simulink model "Testbed_R1"  (R2025a)
settings: Solver=ode1  StartTime=0.0  StopTime=TSTOP_R1  FixedStep=2e-6  RelTol=1e-3
undefined symbols (not defined in the file or in its folder): G_R1, Ion, Lithium, MODE_R1
libraries: spsSeriesRLCBranchLib x8, simulink x4, spsGroundLib x4, spsMosfetLib x4, spsControlledVoltageSourceLib x3, spsCurrentMeasurementLib x3, spsVoltageMeasurementLib x3, spsBatteryLib x1, spsThreePhaseSeriesRLCBranchLib x1, spsThreePhaseVIMeasurementLib x1, spsPVArrayLib x1, spsPWMGenerator2LevelLib x1
settings Model: Creator=ASUS  LastModifiedBy=ASUS
settings DataIOCC: SaveOutput=off  SignalLogging=off  SaveTime=off

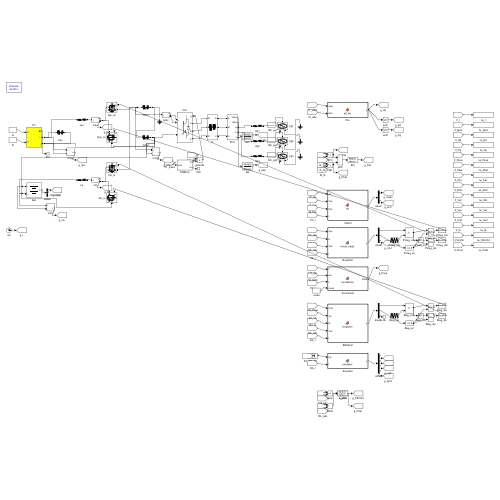
[thumbnail: Simulink's stored preview of the top-level diagram]
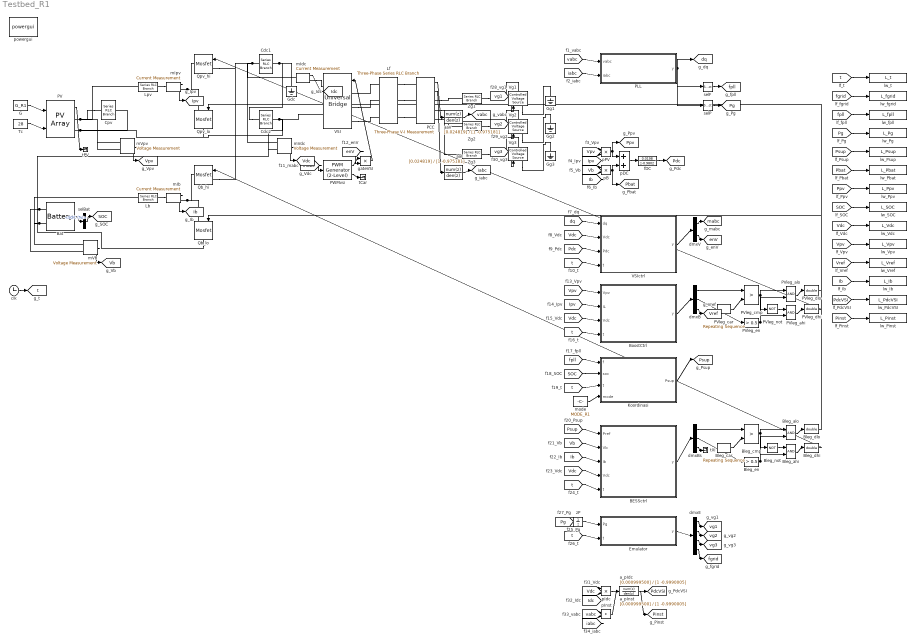
== system Testbed_R1 ==
  BESSctrl : MATLAB Function  TreatAsAtomicUnit=on
  Bat : spsBatteryLib/Battery  BatType=Lithium-Ion  NomV=400  NomQ=150  SOC=SOC0_R1  Batt_Tr=30  PresetModel=on  MaxQ=150  MinV=300  FullV=465.5949  Dis_rate=65.2174  R=0.026667  Normal_OP=135.6522  expZone="[432.1543      7.369565]"
  Bleg_ahi : Logic  AllPortsSameDT=off  OutDataTypeStr=boolean
  Bleg_alo : Logic  AllPortsSameDT=off  OutDataTypeStr=boolean
  Bleg_car : simulink/Sources/Repeating Sequence  rep_seq_t=[0 1e-4 2e-4]  rep_seq_y=[0 1 0]
  Bleg_cmp : RelationalOperator  Operator=>  OutDataTypeStr=boolean  RndMeth=Simplest  InputSameDT=off
  Bleg_dhi : DataTypeConversion  OutDataTypeStr=double  SaturateOnIntegerOverflow=off  RndMeth=Floor
  Bleg_dlo : DataTypeConversion  OutDataTypeStr=double  SaturateOnIntegerOverflow=off  RndMeth=Floor
  Bleg_en : simulink/Logic and Bit Operations/Compare To Constant  relop=>  const=0.5  OutDataTypeStr=boolean
  Bleg_not : Logic  Operator=NOT  AllPortsSameDT=off  OutDataTypeStr=boolean
  BoostCtrl : MATLAB Function  TreatAsAtomicUnit=on
  Cdc1 : spsSeriesRLCBranchLib/Series RLC Branch  LConnTagsString=__new0  RConnTagsString=__new0  BranchType=RC  Resistance=1e-3  Inductance=0  SetiL0=off  InitialCurrent=0  Capacitance=20e-3  Setx0=on  InitialVoltage=400  Measurements=None
  Cdc2 : spsSeriesRLCBranchLib/Series RLC Branch  LConnTagsString=__new0  RConnTagsString=__new0  BranchType=RC  Resistance=1e-3  Inductance=0  SetiL0=off  InitialCurrent=0  Capacitance=20e-3  Setx0=on  InitialVoltage=400  Measurements=None
  Cpv : spsSeriesRLCBranchLib/Series RLC Branch  LConnTagsString=__new0  RConnTagsString=__new0  BranchType=RC  Resistance=1e-3  Inductance=0  SetiL0=off  InitialCurrent=0  Capacitance=2e-3  Setx0=on  InitialVoltage=350  Measurements=None
  Emulator : MATLAB Function  TreatAsAtomicUnit=on
  G : Constant  Value=G_R1
  Gdc : spsGroundLib/Ground  LConnTagsString=a
  Gg1 : spsGroundLib/Ground  LConnTagsString=a
  Gg2 : spsGroundLib/Ground  LConnTagsString=a
  Gg3 : spsGroundLib/Ground  LConnTagsString=a
  Koordinasi : MATLAB Function  TreatAsAtomicUnit=on
  Lb : spsSeriesRLCBranchLib/Series RLC Branch  LConnTagsString=__new0  RConnTagsString=__new0  BranchType=RL  Resistance=0.02  Inductance=1e-3  SetiL0=off  InitialCurrent=0  Capacitance=0  Setx0=off  InitialVoltage=0  Measurements=None
  Lf : spsThreePhaseSeriesRLCBranchLib/Three-Phase Series RLC Branch  LConnTagsString=A|B|C  RConnTagsString=A|B|C  BranchType=RL  Resistance=0.01  Inductance=1.5e-3  Capacitance=1e-6  Measurements=None
  Lpv : spsSeriesRLCBranchLib/Series RLC Branch  LConnTagsString=__new0  RConnTagsString=__new0  BranchType=RL  Resistance=5e-3  Inductance=2e-3  SetiL0=off  InitialCurrent=0  Capacitance=0  Setx0=off  InitialVoltage=0  Measurements=None
  PCC : spsThreePhaseVIMeasurementLib/Three-Phase V-I Measurement  VoltageMeasurement=phase-to-ground  SetLabelV=off  LabelV=Vabc  Vpu=off  VpuLL=off  CurrentMeasurement=yes  SetLabelI=off  LabelI=Iabc  Ipu=off  Pbase=100e6  Vbase=500e3  OutputType=Complex  PhasorSimulation=off  PSBequivalent=0
  PLL : MATLAB Function  TreatAsAtomicUnit=on
  PV : spsPVArrayLib/PV Array  Npar=40  Nser=7  PlotType=array @ 1000 W/m2 & specified temperatures  S_vec="[ 1000  500  100 ]"  Temp_C_vec=[ 0 15 25 35 50]  ModuleName=User-defined  PlotWhenSelected=off  Pm=349.972  Ncell=96  Voc=51.7  Isc=8.65  Vm=43.1  Im=8.12  beta_Voc_pc=-0.37  alpha_Isc_pc=0.07  beta_Voc=-0.19129  alpha_Isc=0.006055  IL=8.6554  I0=4.1764e-10  nI=0.88295  Rsh=412.0293  Rs=0.25518  RobustModel=off  RobustCellTemperature=313.3991  BAL=on  Tc=1e-6  Tfilter=5e-5
  PVleg_ahi : Logic  AllPortsSameDT=off  OutDataTypeStr=boolean
  PVleg_alo : Logic  AllPortsSameDT=off  OutDataTypeStr=boolean
  PVleg_car : simulink/Sources/Repeating Sequence  rep_seq_t=[0 1e-4 2e-4]  rep_seq_y=[0 1 0]
  PVleg_cmp : RelationalOperator  Operator=>  OutDataTypeStr=boolean  RndMeth=Simplest  InputSameDT=off
  PVleg_dhi : DataTypeConversion  OutDataTypeStr=double  SaturateOnIntegerOverflow=off  RndMeth=Floor
  PVleg_dlo : DataTypeConversion  OutDataTypeStr=double  SaturateOnIntegerOverflow=off  RndMeth=Floor
  PVleg_en : simulink/Logic and Bit Operations/Compare To Constant  relop=>  const=0.5  OutDataTypeStr=boolean
  PVleg_not : Logic  Operator=NOT  AllPortsSameDT=off  OutDataTypeStr=boolean
  PWMvsi : spsPWMGenerator2LevelLib/PWM Generator (2-Level)  ModulatorType=Three-phase bridge (6 pulses)  ModulatorMode=Unsynchronized  Fc=5000  Pc=0  nF=10000  MinMax="[ -1  1 ]"  SamplingTechnique=Natural  ModulatingSignals=off  m=0.438786204584116  Freq=50  Phase=0  Ts=2e-6  ShowCarrierOutport=on
  Qb_hi : spsMosfetLib/Mosfet  Ron=1e-3  Lon=0  Rd=0.01  Vfd=0  IC=0  Rs=1e5  Cs=inf  Measurements=off
  Qb_lo : spsMosfetLib/Mosfet  Ron=1e-3  Lon=0  Rd=0.01  Vfd=0  IC=0  Rs=1e5  Cs=inf  Measurements=off
  Qpv_hi : spsMosfetLib/Mosfet  Ron=1e-3  Lon=0  Rd=0.01  Vfd=0  IC=0  Rs=1e5  Cs=inf  Measurements=off
  Qpv_lo : spsMosfetLib/Mosfet  Ron=1e-3  Lon=0  Rd=0.01  Vfd=0  IC=0  Rs=1e5  Cs=inf  Measurements=off
  Tc : Constant  Value=28
  VSI : spsUniversalBridgeLib/Universal Bridge  Arms=3  SnubberResistance=1e5  SnubberCapacitance=inf  Device=IGBT / Diodes  Ron=2.5e-3  Lon=0  ForwardVoltages="[  2.2  1.5  ]"  ForwardVoltage=0  GTOparameters=[ 10e-6 , 20e-6 ]  IGBTparameters=[ 1e-6 , 2e-6 ]  Measurements=None  Measurements_2=None  converterType=Rectifier
  VSIctrl : MATLAB Function  TreatAsAtomicUnit=on
  Vg1 : spsControlledVoltageSourceLib/Controlled Voltage Source  Initialize=off  Source_Type=AC  Amplitude=0  Phase=0  Frequency=0  Measurements=None
  Vg2 : spsControlledVoltageSourceLib/Controlled Voltage Source  Initialize=off  Source_Type=AC  Amplitude=0  Phase=0  Frequency=0  Measurements=None
  Vg3 : spsControlledVoltageSourceLib/Controlled Voltage Source  Initialize=off  Source_Type=AC  Amplitude=0  Phase=0  Frequency=0  Measurements=None
  Zg1 : spsSeriesRLCBranchLib/Series RLC Branch  LConnTagsString=__new0  RConnTagsString=__new0  BranchType=RL  Resistance=0.05  Inductance=0.5e-3  SetiL0=off  InitialCurrent=0  Capacitance=0  Setx0=off  InitialVoltage=0  Measurements=None
  Zg2 : spsSeriesRLCBranchLib/Series RLC Branch  LConnTagsString=__new0  RConnTagsString=__new0  BranchType=RL  Resistance=0.05  Inductance=0.5e-3  SetiL0=off  InitialCurrent=0  Capacitance=0  Setx0=off  InitialVoltage=0  Measurements=None
  Zg3 : spsSeriesRLCBranchLib/Series RLC Branch  LConnTagsString=__new0  RConnTagsString=__new0  BranchType=RL  Resistance=0.05  Inductance=0.5e-3  SetiL0=off  InitialCurrent=0  Capacitance=0  Setx0=off  InitialVoltage=0  Measurements=None
  a_pIdc : DiscreteTransferFcn  Numerator=[0.000999500]  Denominator=[1 -0.9990005]  SampleTime=2e-5
  a_pInst : DiscreteTransferFcn  Numerator=[0.000999500]  Denominator=[1 -0.9990005]  SampleTime=2e-5
  aaI : DiscreteFilter  Numerator=[0.024819]  Denominator=[1 -0.975181]  SampleTime=2e-6
  aaV : DiscreteFilter  Numerator=[0.024819]  Denominator=[1 -0.975181]  SampleTime=2e-6
  clk : Clock
  dmxB : Demux  Outputs=3
  dmxBs : Demux  Outputs=3
  dmxE : Demux
  dmxV : Demux  Outputs=[3 1]
  fDC : DiscreteTransferFcn  Numerator=[0.0198]  Denominator=[1 -0.9802]  SampleTime=1e-4
  gateVSI : Product
  lw_Ib : ToWorkspace  VariableName=L_Ib  SampleTime=1e-3
  lw_Pbat : ToWorkspace  VariableName=L_Pbat  SampleTime=1e-3
  lw_PdcVSI : ToWorkspace  VariableName=L_PdcVSI  SampleTime=1e-3
  lw_Pg : ToWorkspace  VariableName=L_Pg  SampleTime=1e-3
  lw_Pinst : ToWorkspace  VariableName=L_Pinst  SampleTime=1e-3
  lw_Ppv : ToWorkspace  VariableName=L_Ppv  SampleTime=1e-3
  lw_Psup : ToWorkspace  VariableName=L_Psup  SampleTime=1e-3
  lw_SOC : ToWorkspace  VariableName=L_SOC  SampleTime=1e-3
  lw_Vdc : ToWorkspace  VariableName=L_Vdc  SampleTime=1e-3
  lw_Vpv : ToWorkspace  VariableName=L_Vpv  SampleTime=1e-3
  lw_Vref : ToWorkspace  VariableName=L_Vref  SampleTime=1e-3
  lw_fgrid : ToWorkspace  VariableName=L_fgrid  SampleTime=1e-3
  lw_fpll : ToWorkspace  VariableName=L_fpll  SampleTime=1e-3
  lw_t : ToWorkspace  VariableName=L_t  SampleTime=1e-3
  mIb : spsCurrentMeasurementLib/Current Measurement  PhasorSimulation=off  OutputType=Complex  PSBequivalent=0
  mIdc : spsCurrentMeasurementLib/Current Measurement  PhasorSimulation=off  OutputType=Complex  PSBequivalent=0
  mIpv : spsCurrentMeasurementLib/Current Measurement  PhasorSimulation=off  OutputType=Complex  PSBequivalent=0
  mVb : spsVoltageMeasurementLib/Voltage Measurement  PhasorSimulation=off  OutputType=Complex  PSBequivalent=0
  mVdc : spsVoltageMeasurementLib/Voltage Measurement  PhasorSimulation=off  OutputType=Complex  PSBequivalent=0
  mVpv : spsVoltageMeasurementLib/Voltage Measurement  PhasorSimulation=off  OutputType=Complex  PSBequivalent=0
  mode : Constant  Value=MODE_R1
  pB : Product
  pDC : Sum
  pIdc : Product
  pInst : DotProduct  OutDataTypeStr=Inherit: Inherit via internal rule
  pPV : Product
  powergui : spspowerguiLib/powergui  Priority=1  SimulationMode=Discrete  SampleTime=2e-6  frequency=60  Iterations=50  frequencyindice=60  Pbase=100e6  ErrMax=1e-4  UnitsV=kV  UnitsW=MW  buscounter=0  FunctionMessages=off  echomessages=off  EnableUseOfTLC=off  CurrentSourceSwitches=off  DisableSnubberDevices=off  DisableRonSwitches=off  DisableVfSwitches=off  DisplayEquations=off  AutomaticDiscreteSolvers=off  SolverType=Tustin/Backward Euler (TBE)  Interpol=off  ExternalGateDelay=off  methode=off  Ts=100  x0status=blocks  SPID=on  SwTol=0  HookPort=off  NonlinearTolerance=1e-4  nMaxIteration=100  ContinueOnMaxIteration=off  RestoreLinks=warning  ResistiveCurrentMeasurement=off  Frange=[0:2:500]  Ylog=off  Xlog=on  ShowGrid=off  save=off  variable=ZData  structure=0  ZoomFFT=off  StartTime=0.0  cycles=1  DisplayStyle=1  fundamental=60  FreqAxis=off  MaxFrequency=1000  frequencyindicesteady=1  RmsSteady=1  display=off
  selBat : BusSelector  OutputSignals=SOC (%)
  selF : Selector  InputPortWidth=8  IndexOptions=Index vector (dialog)  Indices=2  OutputSizes=1
  selP : Selector  InputPortWidth=8  IndexOptions=Index vector (dialog)  Indices=7  OutputSizes=1
  tCar : Terminator
  tPV : Terminator
  tXi : Terminator
  zP : UnitDelay  SampleTime=1e-4  HasFrameUpgradeWarning=on
  tag scope: Ib=global, Idc=global, Ipv=global, Pbat=global, Pdc=global, PdcVSI=global, Pg=global, Pinst=global, Ppv=global, Psup=global, SOC=global, Vb=global, Vdc=global, Vpv=global, Vref=global, dq=global, enV=global, fgrid=global, fpll=global, iabc=global, mabc=global, t=global, vabc=global, vg1=global, vg2=global, vg3=global
  wires:
  G/1 -> PV/1
  Tc/1 -> PV/2
  PV/1 -> tPV/1
  PWMvsi/2 -> tCar/1
  PWMvsi/1 -> gateVSI/1
  gateVSI/1 -> VSI/1
  clk/1 -> [t]
  mVpv/1 -> [Vpv]
  mIpv/1 -> [Ipv]
  mVdc/1 -> [Vdc]
  mVb/1 -> [Vb]
  mIb/1 -> [Ib]
  PCC/1 -> aaV/1
  PCC/2 -> aaI/1
  aaV/1 -> [vabc]
  aaI/1 -> [iabc]
  Bat/1 -> selBat/1
  selBat/1 -> [SOC]  "<SOC (%)>"
  [vabc] -> PLL/1(vabc)
  [iabc] -> PLL/2(iabc)
  PLL/1(y) -> [dq], selF/1, selP/1
  selF/1 -> [fpll]
  selP/1 -> [Pg]
  [Vpv] -> pPV/1
  [Ipv] -> pPV/2
  [Vb] -> pB/1
  [Ib] -> pB/2
  pPV/1 -> pDC/1, [Ppv]
  pB/1 -> pDC/2, [Pbat]
  pDC/1 -> fDC/1
  fDC/1 -> [Pdc]
  [dq] -> VSIctrl/1(dq)
  [Vdc] -> VSIctrl/2(Vdc)
  [Pdc] -> VSIctrl/3(Pdc)
  [t] -> VSIctrl/4(t)
  VSIctrl/1(y) -> dmxV/1
  dmxV/1 -> [mabc]
  dmxV/2 -> [enV]
  [mabc] -> PWMvsi/1
  [enV] -> gateVSI/2
  [Vpv] -> BoostCtrl/1(Vpv)
  [Ipv] -> BoostCtrl/2(IL)
  [Vdc] -> BoostCtrl/3(Vdc)
  [t] -> BoostCtrl/4(t)
  BoostCtrl/1(y) -> dmxB/1
  dmxB/3 -> [Vref]
  dmxB/1 -> PVleg_cmp/1
  PVleg_car/1 -> PVleg_cmp/2
  dmxB/2 -> PVleg_en/1
  PVleg_cmp/1 -> PVleg_alo/1, PVleg_not/1
  PVleg_en/1 -> PVleg_alo/2, PVleg_ahi/2
  PVleg_not/1 -> PVleg_ahi/1
  PVleg_alo/1 -> PVleg_dlo/1
  PVleg_ahi/1 -> PVleg_dhi/1
  PVleg_dlo/1 -> Qpv_lo/1
  PVleg_dhi/1 -> Qpv_hi/1
  [fpll] -> Koordinasi/1(f)
  [SOC] -> Koordinasi/2(soc)
  [t] -> Koordinasi/3(t)
  mode/1 -> Koordinasi/4(mode)
  Koordinasi/1(Psup) -> [Psup]
  [Psup] -> BESSctrl/1(Pref)
  [Vb] -> BESSctrl/2(Vb)
  [Ib] -> BESSctrl/3(Ib)
  [Vdc] -> BESSctrl/4(Vdc)
  [t] -> BESSctrl/5(t)
  BESSctrl/1(y) -> dmxBs/1
  dmxBs/3 -> tXi/1
  dmxBs/1 -> Bleg_cmp/1
  Bleg_car/1 -> Bleg_cmp/2
  dmxBs/2 -> Bleg_en/1
  Bleg_cmp/1 -> Bleg_alo/1, Bleg_not/1
  Bleg_en/1 -> Bleg_alo/2, Bleg_ahi/2
  Bleg_not/1 -> Bleg_ahi/1
  Bleg_alo/1 -> Bleg_dlo/1
  Bleg_ahi/1 -> Bleg_dhi/1
  Bleg_dlo/1 -> Qb_lo/1
  Bleg_dhi/1 -> Qb_hi/1
  [t] -> Emulator/2(t)
  [Pg] -> zP/1
  zP/1 -> Emulator/1(Pg)
  Emulator/1(y) -> dmxE/1
  dmxE/1 -> [vg1]
  [vg1] -> Vg1/1
  dmxE/2 -> [vg2]
  [vg2] -> Vg2/1
  dmxE/3 -> [vg3]
  [vg3] -> Vg3/1
  dmxE/4 -> [fgrid]
  [Vdc] -> pIdc/1
  mIdc/1 -> [Idc]
  [Idc] -> pIdc/2
  [vabc] -> pInst/1
  [iabc] -> pInst/2
  pIdc/1 -> a_pIdc/1
  pInst/1 -> a_pInst/1
  a_pIdc/1 -> [PdcVSI]
  a_pInst/1 -> [Pinst]
  [t] -> lw_t/1
  [fgrid] -> lw_fgrid/1
  [fpll] -> lw_fpll/1
  [Pg] -> lw_Pg/1
  [Psup] -> lw_Psup/1
  [Pbat] -> lw_Pbat/1
  [Ppv] -> lw_Ppv/1
  [SOC] -> lw_SOC/1
  [Vdc] -> lw_Vdc/1
  [Vpv] -> lw_Vpv/1
  [Vref] -> lw_Vref/1
  [Ib] -> lw_Ib/1
  [PdcVSI] -> lw_PdcVSI/1
  [Pinst] -> lw_Pinst/1
  connections:
  Cpv/LConn1 -- PV/RConn1 -- mVpv/LConn1 -- Lpv/LConn1
  Cpv/RConn1 -- PV/RConn2 -- mVpv/LConn2 -- Cdc2/RConn1 -- Qpv_lo/RConn1 -- mVdc/LConn2 -- mVb/LConn2 -- Qb_lo/RConn1 -- Bat/LConn2 -- VSI/RConn2
  Lpv/RConn1 -- mIpv/LConn1
  Qpv_lo/LConn1 -- mIpv/RConn1 -- Qpv_hi/RConn1
  Qpv_hi/LConn1 -- mVdc/LConn1 -- Qb_hi/LConn1 -- Cdc1/LConn1 -- mIdc/LConn1
  Cdc2/LConn1 -- Cdc1/RConn1 -- Gdc/LConn1
  Bat/LConn1 -- mVb/LConn1 -- Lb/LConn1
  Lb/RConn1 -- mIb/LConn1
  Qb_lo/LConn1 -- mIb/RConn1 -- Qb_hi/RConn1
  mIdc/RConn1 -- VSI/RConn1
  VSI/LConn1 -- Lf/LConn1
  Lf/RConn1 -- PCC/LConn1
  PCC/RConn1 -- Zg1/LConn1
  Zg1/RConn1 -- Vg1/RConn1
  Vg1/LConn1 -- Gg1/LConn1
  VSI/LConn2 -- Lf/LConn2
  Lf/RConn2 -- PCC/LConn2
  PCC/RConn2 -- Zg2/LConn1
  Zg2/RConn1 -- Vg2/RConn1
  Vg2/LConn1 -- Gg2/LConn1
  VSI/LConn3 -- Lf/LConn3
  Lf/RConn3 -- PCC/LConn3
  PCC/RConn3 -- Zg3/LConn1
  Zg3/RConn1 -- Vg3/RConn1
  Vg3/LConn1 -- Gg3/LConn1

== matlab function Testbed_R1/VSIctrl ==
  settings: updateMethod=DISCRETE  sampleTime=0.0001
  data: dq input; y output; Vdc input; Pdc input; t input
function y = vsi(dq, Vdc, Pdc, t)
% Kendali arus dq VSI 2-level + pengatur tegangan DC (Ts 1e-4).
% dq = [theta; f; vd; vq; id; iq; P; Q] dari pll_dq. Pdc = P_PV + P_BESS terukur (umpan maju).
% Keluaran y = [ma; mb; mc; en]  (indeks modulasi, [-1, 1]).
persistent xd xq xv
if isempty(xd), xd = 0; xq = 0; xv = 0; end
Ts = 1e-4; L = 1.5e-3; VREF = 800; T_EN = 0.02; IMAX = 320;
th = dq(1); w = 2*pi*dq(2); vd = dq(3); vq = dq(4); id = dq(5); iq = dq(6);
en = double(t >= T_EN);
% pengatur tegangan DC: Vdc di atas acuan -> ekspor lebih banyak
ev = Vdc - VREF;
xv = min(max(xv + en*35*Ts*ev, -IMAX), IMAX);
id_ff = Pdc / (1.5*max(vd, 200));
id_ref = min(max(id_ff + 1.5*ev + xv, -IMAX), IMAX);
iq_ref = 0;                                          % faktor daya satu
% arus
Kp = 2.83; Ki = 300;
ed_ = id_ref - id; eq_ = iq_ref - iq;
xd = min(max(xd + en*Ki*Ts*ed_, -200), 200);
xq = min(max(xq + en*Ki*Ts*eq_, -200), 200);
ud = vd - w*L*iq + Kp*ed_ + xd;
uq = vq + w*L*id + Kp*eq_ + xq;
if en == 0, xd = 0; xq = 0; xv = 0; ud = vd; uq = vq; end
thm = th + 1.5*Ts*w;                                 % kompensasi tunda komputasi + PWM
c = cos(thm); s = sin(thm);
ua = c*ud - s*uq; ub = s*ud + c*uq;
uabc = [ua; -0.5*ua + sqrt(3)/2*ub; -0.5*ua - sqrt(3)/2*ub];
m = uabc / (max(Vdc, 100)/2);
m = min(max(m, -1), 1);
y = [m; en];
end

== matlab function Testbed_R1/PLL ==
  settings: updateMethod=DISCRETE  sampleTime=0.0001
  data: vabc input; y output; iabc input
function y = pll_dq(vabc, iabc)
% PLL kerangka-sinkron (SRF) + transformasi dq (Ts 1e-4). Arus positif = inverter -> jaringan.
% Keluaran y = [theta; f; vd; vq; id; iq; P; Q]
persistent th w xi
if isempty(th), th = 0; w = 2*pi*50; xi = 0; end
Ts = 1e-4; W0 = 2*pi*50; VPK = 400*sqrt(2/3);
Kp = 176; Ki = 15791;                      % omega_n = 2*pi*20, zeta = 0,7 (ternormalisasi)
va = 2/3*(vabc(1) - 0.5*vabc(2) - 0.5*vabc(3));
vb = 2/3*(sqrt(3)/2)*(vabc(2) - vabc(3));
ia = 2/3*(iabc(1) - 0.5*iabc(2) - 0.5*iabc(3));
ib = 2/3*(sqrt(3)/2)*(iabc(2) - iabc(3));
c = cos(th); s = sin(th);
vd =  c*va + s*vb;  vq = -s*va + c*vb;
id =  c*ia + s*ib;  iq = -s*ia + c*ib;
e = vq / VPK;
xi = xi + Ki*Ts*e;
w = W0 + Kp*e + xi;
th = th + w*Ts;
if th > 2*pi, th = th - 2*pi; end
P = 1.5*(vd*id + vq*iq);  Q = 1.5*(vq*id - vd*iq);
y = [th; w/(2*pi); vd; vq; id; iq; P; Q];
end

== matlab function Testbed_R1/BoostCtrl ==
  settings: updateMethod=DISCRETE  sampleTime=0.0002
  data: Vpv input; y output; IL input; Vdc input; t input
function y = boost_mppt(Vpv, IL, Vdc, t)
% Boost sinkron PV: MPPT P&O (langkah 2 V tiap 40 ms) -> loop tegangan PV -> loop arus induktor.
% Ts 2e-4, disampel di lembah pembawa segitiga 5 kHz. Keluaran y = [d; en; Vref].
persistent Vref dir Pacc nacc Pprev k xv xi
if isempty(Vref)
    Vref = 0.85*7*51.7; dir = -1; Pacc = 0; nacc = 0; Pprev = 0; k = 0; xv = 0; xi = 0;
end
Ts = 2e-4; T_EN = 0.05; STEP = 2.0; N_MPPT = 200;    % 200 x 2e-4 = 40 ms
VMIN = 0.60*7*51.7; VMAX = 0.95*7*51.7;
en = double(t >= T_EN);
if en > 0
    Pacc = Pacc + Vpv*IL; nacc = nacc + 1; k = k + 1;
    if k >= N_MPPT
        P = Pacc / nacc;
        if P < Pprev, dir = -dir; end
        Pprev = P; Vref = min(max(Vref + dir*STEP, VMIN), VMAX);
        Pacc = 0; nacc = 0; k = 0;
    end
end
% loop tegangan PV: Vpv di atas acuan -> tarik arus lebih besar
ev = Vpv - Vref;
xv = min(max(xv + en*200*Ts*ev, -400), 400);
Iref = min(max(1.0*ev + xv, 0), 400);
% loop arus induktor (sama dengan loop BESS): V_L = Vpv - (1-d) Vdc
e = Iref - IL;
xi = min(max(xi + en*720*Ts*e, -300), 300);
u = 3.8*e + xi;
if en == 0, xv = 0; xi = 0; end
d = 1 - (Vpv - u) / max(Vdc, 1);
d = min(max(d, 0.02), 0.98);
y = [d; en; Vref];
end

== matlab function Testbed_R1/Koordinasi ==
  settings: updateMethod=DISCRETE  sampleTime=0.0001
  data: f input; Psup output; soc input; t input; mode input
function Psup = koordinasi(f, soc, t, mode)
% Koordinasi dukungan frekuensi (Ts 1e-4), cermin python/fullmodel.py.
% mode 0 = tanpa dukungan, 1 = skema usulan (knee), 2 = relai statis naskah,
% 3 = relai FFR 49,7 Hz (h 0,006, M 0,15), 9 = uji: 20 kW konstan mulai 0,6 s. Keluaran: P_sup [W] (positif = ekspor).
persistent Dwf
if isempty(Dwf), Dwf = 0; end
Ts = 1e-4; tau = 0.02; S = 100e3; T_ON = 1.0;
Dw = (f - 50) / 50;
rocof = (Dw - Dwf) / tau;
Dwf = Dwf + Ts * (Dw - Dwf) / tau;
s = soc / 100;
phi_d = min(max((s - 0.20) / 0.05, 0), 1);
phi_c = min(max((0.90 - s) / 0.05, 0), 1);
P = 0;
if mode == 1
    Pvic = -(1.0045 * Dwf + 0.0317 * rocof);
    a = 1 / (1 + 47.483 * abs(Dwf) + 1.0 * abs(rocof));
    raw = 0.2497 * tanh(45.797 * (-Dwf));
    if raw >= 0, Pb = raw * phi_d; else, Pb = raw * phi_c; end
    P = (1 - a) * Pvic + Pb;
elseif mode == 2 || mode == 3
    if mode == 2, h = 0.02; M = 0.40; else, h = 0.006; M = 0.15; end
    Pvic = -(0.5 * Dwf + 0.1 * rocof);
    st = 0;
    if Dwf < -h, st = 1; elseif Dwf > h, st = -1; end
    if st > 0, Pb = M * phi_d; elseif st < 0, Pb = -M * phi_c; else, Pb = 0; end
    P = Pvic + Pb;
end
if t < T_ON, P = 0; end
if mode == 9 && t >= 0.6, P = 20e3 / S; end   % uji polaritas/aliran daya
Psup = P * S;
end

== matlab function Testbed_R1/BESSctrl ==
  settings: updateMethod=DISCRETE  sampleTime=0.0002
  data: Pref input; y output; Vb input; Ib input; Vdc input; t input
function y = looparus(Pref, Vb, Ib, Vdc, t)
% Loop arus konverter BESS dua arah (Ts 2e-4, disampel di lembah pembawa segitiga 5 kHz
% sehingga sampel = arus rata-rata; versi 2e-5 dengan pembawa gigi gergaji ber-aliasing). Ib positif = pelepasan (baterai -> DC-link);
% tanda dicek 20 Okt: duty 0,98 menghasilkan Ib = +2800 A (hubung singkat lewat Q_lo).
% Boost rata-rata: V_L = Vb - (1-d) Vdc  ->  d = 1 - (Vb - u)/Vdc, u = PI(Iref - Ib).
% Kedua gate dimatikan (en = 0) sampai T_EN agar DC-link selesai start-up.
persistent xi
if isempty(xi), xi = 0; end
Ts = 2e-4; Kp = 1.9; Ki = 360; IMAX = 120; T_EN = 0.05;
en = double(t >= T_EN);
Iref = Pref / max(Vb, 300);
Iref = min(max(Iref, -IMAX), IMAX);
e = Iref - Ib;
if en == 0, xi = 0; end
u = Kp * e + xi;
xi = min(max(xi + en * Ki * Ts * e, -300), 300);
d = 1 - (Vb - u) / max(Vdc, 1);
d = min(max(d, 0.02), 0.98);
y = [d; en; xi];
end

== matlab function Testbed_R1/Emulator ==
  settings: updateMethod=DISCRETE  sampleTime=1e-05
  data: Pg input; y output; t input
function y = emulator(Pg, t)
% Emulator jaringan agregat (Ts 1e-5): tegangan tiga fasa dengan frekuensi dari persamaan ayun
%   2H dDw/dt = (P_eksp - P_jadwal)/S_g - dP_L(t) - D Dw     (pu pada S_g)
% P_eksp = P terukur di PCC dari pll_dq (positif = ekspor), difilter 20 ms.
% Ayun dibekukan sampai T_SCHED (inisialisasi MPPT); P_jadwal = P_eksp rerata 0,3 s terakhir.
% Keluaran y = [va; vb; vc; f_grid].
persistent th Dw Pf Pacc nacc Psch
if isempty(th), th = 0; Dw = 0; Pf = 0; Pacc = 0; nacc = 0; Psch = 0; end
Ts = 1e-5; S = 100e3; H = 2.0; D = 1.0; DPL = 0.10;
T_SCHED = 1.5; T_EVT = 2.0; VPK = 400 * sqrt(2/3);
Pf = Pf + Ts * (Pg - Pf) / 0.02;
if t >= T_SCHED - 0.3 && t < T_SCHED
    Pacc = Pacc + Pf; nacc = nacc + 1;
end
if t >= T_SCHED
    if nacc > 0 && Psch == 0, Psch = Pacc / nacc; end
    dist = 0;
    if t >= T_EVT, dist = DPL; end
    Dw = Dw + Ts * ((Pf - Psch) / S - dist - D * Dw) / (2 * H);
    Dw = min(max(Dw, -0.2), 0.2);
end
f = 50 * (1 + Dw);
th = th + Ts * 2 * pi * f;
if th > 2 * pi, th = th - 2 * pi; end
y = [VPK * sin(th); VPK * sin(th - 2*pi/3); VPK * sin(th + 2*pi/3); f];
end
